simulink model "Residential_grid4"  (R2026a)
settings: Solver=VariableStepAuto  StopTime=365*24*3600
undefined symbols (not defined in the file): evCharge, load1, load2, load3, load4, Solar, Wind
libraries: fl_lib x132, nesl_utility x61
(part 1 of 3)
settings Model: Creator=xiaos  LastModifiedBy=hiro
settings DebuggingCC: SaveWithParameterizedLinksMsg=none
settings SimscapeCC: SimscapeNominalValues="[{\"value\":\"1\",\"unit\":\"A\"},{\"value\":\"1\",\"unit\":\"bar\"},{\"value\":\"1\",\"unit\":\"cm^2\"},{\"value\":\"1\",\"unit\":\"cm^3/s\"},{\"value\":\"1\",\"unit\":\"kJ/kg\"},{\"value\":\"1\",\"unit\":\"kW\"},{\"value\":\"1\",\"unit\":\"l\"},{\"value\":\"1\",\"unit\":\"N\"},{\"value\":\"1\",\"unit\":\"N*m\"},{\"value\":\"1\",\"unit\":\"V\"}]"  SimscapeLogType=none  SimscapeLogDataHistory=5000.0

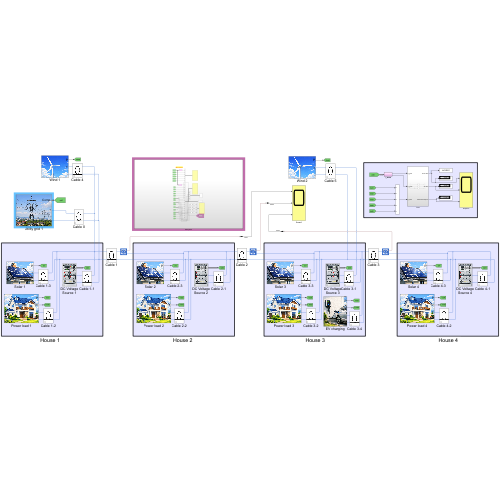
[thumbnail: Simulink's stored preview of the top-level diagram]
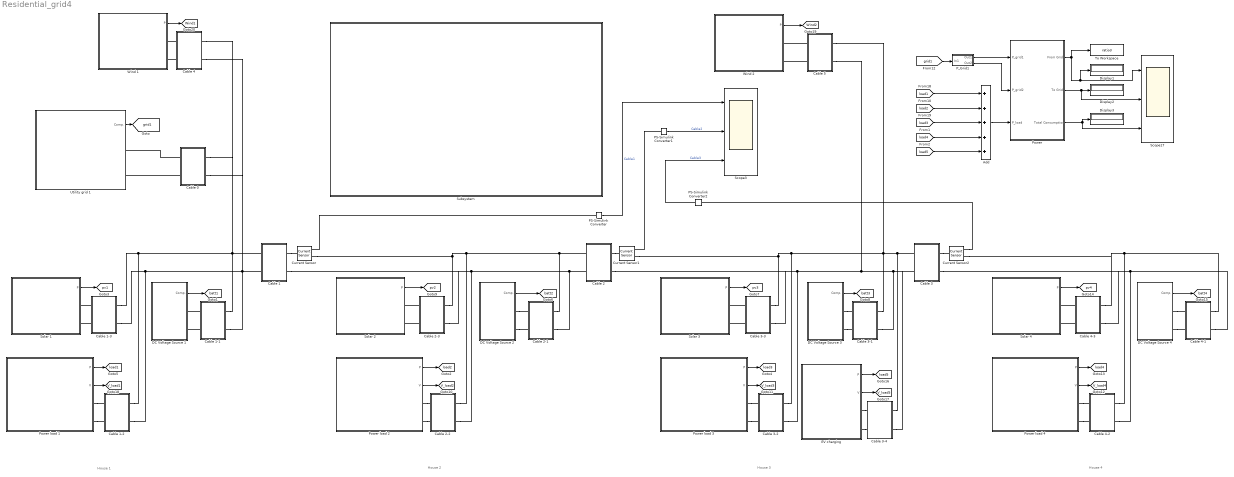
== system Residential_grid4 ==
  note: House 1
  note: House 2
  note: House 3
  note: House 4
  Add : Sum  Inputs=+++++
  Cable 0 : Subsystem  mask{intR=3.01, L=20, SQ=SQ,  rc,  Ampacity}
      mask prompts: intR "Conductor resistance: rc (Ω/km)"; L "Length: L (m)"; SQ "For reference: CV cable constants"
      mask TypeOptions SQ: SQ,  rc,  Ampacity | 2 (mm2),  12 (Ω/km),  28 (A) | 3.5 (mm2),  6.76 (Ω/km),  39 (A) | 5.5 (mm2),  4.34 (Ω/km),  52 (A) | 8 (mm2),  3.01 (Ω/km),   65 (A) | 14 (mm2),  1.71 (Ω/km),  91 (A) | 22 (mm2),  1.08 (Ω/km),  120 (A) | 38 (mm2),  0.626 (Ω/km),  170 (A) | 60 (mm2),  0.397 (Ω/km),  225 (A) | 100 (mm2),  0.239 (Ω/km),  310 (A) | 150 (mm2),  0.16 (Ω/km),  400 (A) | 200 (mm2),  0.121 (Ω/km),  485 (A) | 250 (mm2),  0.0985 (Ω/km),  560 (A) | 325 (mm2),  0.077 (Ω/km),  660 (A)
      mask DialogControl DescTextVar Prompt: 2-Core CV Cable
      mask Display: image('cable_1.png');
  Cable 1 : Subsystem  mask{intR=3.01, L=50, SQ=SQ,  rc,  Ampacity}
      mask prompts: intR "Conductor resistance: rc (Ω/km)"; L "Length: L (m)"; SQ "For reference: CV cable constants"
      mask TypeOptions SQ: SQ,  rc,  Ampacity | 2 (mm2),  12 (Ω/km),  28 (A) | 3.5 (mm2),  6.76 (Ω/km),  39 (A) | 5.5 (mm2),  4.34 (Ω/km),  52 (A) | 8 (mm2),  3.01 (Ω/km),   65 (A) | 14 (mm2),  1.71 (Ω/km),  91 (A) | 22 (mm2),  1.08 (Ω/km),  120 (A) | 38 (mm2),  0.626 (Ω/km),  170 (A) | 60 (mm2),  0.397 (Ω/km),  225 (A) | 100 (mm2),  0.239 (Ω/km),  310 (A) | 150 (mm2),  0.16 (Ω/km),  400 (A) | 200 (mm2),  0.121 (Ω/km),  485 (A) | 250 (mm2),  0.0985 (Ω/km),  560 (A) | 325 (mm2),  0.077 (Ω/km),  660 (A)
      mask DialogControl DescTextVar Prompt: 2-Core CV Cable
      mask Display: image('cable_2.png');
  Cable 1-1 : Subsystem  mask{intR=3.01, L=5, SQ=SQ,  rc,  Ampacity}
      mask prompts: intR "Conductor resistance: rc (Ω/km)"; L "Length: L (m)"; SQ "For reference: CV cable constants"
      mask TypeOptions SQ: SQ,  rc,  Ampacity | 2 (mm2),  12 (Ω/km),  28 (A) | 3.5 (mm2),  6.76 (Ω/km),  39 (A) | 5.5 (mm2),  4.34 (Ω/km),  52 (A) | 8 (mm2),  3.01 (Ω/km),   65 (A) | 14 (mm2),  1.71 (Ω/km),  91 (A) | 22 (mm2),  1.08 (Ω/km),  120 (A) | 38 (mm2),  0.626 (Ω/km),  170 (A) | 60 (mm2),  0.397 (Ω/km),  225 (A) | 100 (mm2),  0.239 (Ω/km),  310 (A) | 150 (mm2),  0.16 (Ω/km),  400 (A) | 200 (mm2),  0.121 (Ω/km),  485 (A) | 250 (mm2),  0.0985 (Ω/km),  560 (A) | 325 (mm2),  0.077 (Ω/km),  660 (A)
      mask DialogControl DescTextVar Prompt: 2-Core CV Cable
      mask Display: image('cable_7.png');
  Cable 1-2 : Subsystem  mask{intR=3.01, L=10, SQ=SQ,  rc,  Ampacity}
      mask prompts: intR "Conductor resistance: rc (Ω/km)"; L "Length: L (m)"; SQ "For reference: CV cable constants"
      mask TypeOptions SQ: SQ,  rc,  Ampacity | 2 (mm2),  12 (Ω/km),  28 (A) | 3.5 (mm2),  6.76 (Ω/km),  39 (A) | 5.5 (mm2),  4.34 (Ω/km),  52 (A) | 8 (mm2),  3.01 (Ω/km),   65 (A) | 14 (mm2),  1.71 (Ω/km),  91 (A) | 22 (mm2),  1.08 (Ω/km),  120 (A) | 38 (mm2),  0.626 (Ω/km),  170 (A) | 60 (mm2),  0.397 (Ω/km),  225 (A) | 100 (mm2),  0.239 (Ω/km),  310 (A) | 150 (mm2),  0.16 (Ω/km),  400 (A) | 200 (mm2),  0.121 (Ω/km),  485 (A) | 250 (mm2),  0.0985 (Ω/km),  560 (A) | 325 (mm2),  0.077 (Ω/km),  660 (A)
      mask DialogControl DescTextVar Prompt: 2-Core CV Cable
      mask Display: image('cable_8.png');
  Cable 1-3 : Subsystem  mask{intR=3.01, L=10, SQ=SQ,  rc,  Ampacity}
      mask prompts: intR "Conductor resistance: rc (Ω/km)"; L "Length: L (m)"; SQ "For reference: CV cable constants"
      mask TypeOptions SQ: SQ,  rc,  Ampacity | 2 (mm2),  12 (Ω/km),  28 (A) | 3.5 (mm2),  6.76 (Ω/km),  39 (A) | 5.5 (mm2),  4.34 (Ω/km),  52 (A) | 8 (mm2),  3.01 (Ω/km),   65 (A) | 14 (mm2),  1.71 (Ω/km),  91 (A) | 22 (mm2),  1.08 (Ω/km),  120 (A) | 38 (mm2),  0.626 (Ω/km),  170 (A) | 60 (mm2),  0.397 (Ω/km),  225 (A) | 100 (mm2),  0.239 (Ω/km),  310 (A) | 150 (mm2),  0.16 (Ω/km),  400 (A) | 200 (mm2),  0.121 (Ω/km),  485 (A) | 250 (mm2),  0.0985 (Ω/km),  560 (A) | 325 (mm2),  0.077 (Ω/km),  660 (A)
      mask DialogControl DescTextVar Prompt: 2-Core CV Cable
      mask Display: image('cable_9.png');
  Cable 2 : Subsystem  mask{intR=3.01, L=50, SQ=SQ,  rc,  Ampacity}
      mask prompts: intR "Conductor resistance: rc (Ω/km)"; L "Length: L (m)"; SQ "For reference: CV cable constants"
      mask TypeOptions SQ: SQ,  rc,  Ampacity | 2 (mm2),  12 (Ω/km),  28 (A) | 3.5 (mm2),  6.76 (Ω/km),  39 (A) | 5.5 (mm2),  4.34 (Ω/km),  52 (A) | 8 (mm2),  3.01 (Ω/km),   65 (A) | 14 (mm2),  1.71 (Ω/km),  91 (A) | 22 (mm2),  1.08 (Ω/km),  120 (A) | 38 (mm2),  0.626 (Ω/km),  170 (A) | 60 (mm2),  0.397 (Ω/km),  225 (A) | 100 (mm2),  0.239 (Ω/km),  310 (A) | 150 (mm2),  0.16 (Ω/km),  400 (A) | 200 (mm2),  0.121 (Ω/km),  485 (A) | 250 (mm2),  0.0985 (Ω/km),  560 (A) | 325 (mm2),  0.077 (Ω/km),  660 (A)
      mask DialogControl DescTextVar Prompt: 2-Core CV Cable
      mask Display: image('cable_3.png');
  Cable 2-1 : Subsystem  mask{intR=3.01, L=5, SQ=SQ,  rc,  Ampacity}
      mask prompts: intR "Conductor resistance: rc (Ω/km)"; L "Length: L (m)"; SQ "For reference: CV cable constants"
      mask TypeOptions SQ: SQ,  rc,  Ampacity | 2 (mm2),  12 (Ω/km),  28 (A) | 3.5 (mm2),  6.76 (Ω/km),  39 (A) | 5.5 (mm2),  4.34 (Ω/km),  52 (A) | 8 (mm2),  3.01 (Ω/km),   65 (A) | 14 (mm2),  1.71 (Ω/km),  91 (A) | 22 (mm2),  1.08 (Ω/km),  120 (A) | 38 (mm2),  0.626 (Ω/km),  170 (A) | 60 (mm2),  0.397 (Ω/km),  225 (A) | 100 (mm2),  0.239 (Ω/km),  310 (A) | 150 (mm2),  0.16 (Ω/km),  400 (A) | 200 (mm2),  0.121 (Ω/km),  485 (A) | 250 (mm2),  0.0985 (Ω/km),  560 (A) | 325 (mm2),  0.077 (Ω/km),  660 (A)
      mask DialogControl DescTextVar Prompt: 2-Core CV Cable
      mask Display: image('cable_10.png');
  Cable 2-2 : Subsystem  mask{intR=3.01, L=10, SQ=SQ,  rc,  Ampacity}
      mask prompts: intR "Conductor resistance: rc (Ω/km)"; L "Length: L (m)"; SQ "For reference: CV cable constants"
      mask TypeOptions SQ: SQ,  rc,  Ampacity | 2 (mm2),  12 (Ω/km),  28 (A) | 3.5 (mm2),  6.76 (Ω/km),  39 (A) | 5.5 (mm2),  4.34 (Ω/km),  52 (A) | 8 (mm2),  3.01 (Ω/km),   65 (A) | 14 (mm2),  1.71 (Ω/km),  91 (A) | 22 (mm2),  1.08 (Ω/km),  120 (A) | 38 (mm2),  0.626 (Ω/km),  170 (A) | 60 (mm2),  0.397 (Ω/km),  225 (A) | 100 (mm2),  0.239 (Ω/km),  310 (A) | 150 (mm2),  0.16 (Ω/km),  400 (A) | 200 (mm2),  0.121 (Ω/km),  485 (A) | 250 (mm2),  0.0985 (Ω/km),  560 (A) | 325 (mm2),  0.077 (Ω/km),  660 (A)
      mask DialogControl DescTextVar Prompt: 2-Core CV Cable
      mask Display: image('cable_11.png');
  Cable 2-3 : Subsystem  mask{intR=3.01, L=10, SQ=SQ,  rc,  Ampacity}
      mask prompts: intR "Conductor resistance: rc (Ω/km)"; L "Length: L (m)"; SQ "For reference: CV cable constants"
      mask TypeOptions SQ: SQ,  rc,  Ampacity | 2 (mm2),  12 (Ω/km),  28 (A) | 3.5 (mm2),  6.76 (Ω/km),  39 (A) | 5.5 (mm2),  4.34 (Ω/km),  52 (A) | 8 (mm2),  3.01 (Ω/km),   65 (A) | 14 (mm2),  1.71 (Ω/km),  91 (A) | 22 (mm2),  1.08 (Ω/km),  120 (A) | 38 (mm2),  0.626 (Ω/km),  170 (A) | 60 (mm2),  0.397 (Ω/km),  225 (A) | 100 (mm2),  0.239 (Ω/km),  310 (A) | 150 (mm2),  0.16 (Ω/km),  400 (A) | 200 (mm2),  0.121 (Ω/km),  485 (A) | 250 (mm2),  0.0985 (Ω/km),  560 (A) | 325 (mm2),  0.077 (Ω/km),  660 (A)
      mask DialogControl DescTextVar Prompt: 2-Core CV Cable
      mask Display: image('cable_12.png');
  Cable 3 : Subsystem  mask{intR=3.01, L=50, SQ=SQ,  rc,  Ampacity}
      mask prompts: intR "Conductor resistance: rc (Ω/km)"; L "Length: L (m)"; SQ "For reference: CV cable constants"
      mask TypeOptions SQ: SQ,  rc,  Ampacity | 2 (mm2),  12 (Ω/km),  28 (A) | 3.5 (mm2),  6.76 (Ω/km),  39 (A) | 5.5 (mm2),  4.34 (Ω/km),  52 (A) | 8 (mm2),  3.01 (Ω/km),   65 (A) | 14 (mm2),  1.71 (Ω/km),  91 (A) | 22 (mm2),  1.08 (Ω/km),  120 (A) | 38 (mm2),  0.626 (Ω/km),  170 (A) | 60 (mm2),  0.397 (Ω/km),  225 (A) | 100 (mm2),  0.239 (Ω/km),  310 (A) | 150 (mm2),  0.16 (Ω/km),  400 (A) | 200 (mm2),  0.121 (Ω/km),  485 (A) | 250 (mm2),  0.0985 (Ω/km),  560 (A) | 325 (mm2),  0.077 (Ω/km),  660 (A)
      mask DialogControl DescTextVar Prompt: 2-Core CV Cable
      mask Display: image('cable_4.png');
  Cable 3-1 : Subsystem  mask{intR=3.01, L=5, SQ=SQ,  rc,  Ampacity}
      mask prompts: intR "Conductor resistance: rc (Ω/km)"; L "Length: L (m)"; SQ "For reference: CV cable constants"
      mask TypeOptions SQ: SQ,  rc,  Ampacity | 2 (mm2),  12 (Ω/km),  28 (A) | 3.5 (mm2),  6.76 (Ω/km),  39 (A) | 5.5 (mm2),  4.34 (Ω/km),  52 (A) | 8 (mm2),  3.01 (Ω/km),   65 (A) | 14 (mm2),  1.71 (Ω/km),  91 (A) | 22 (mm2),  1.08 (Ω/km),  120 (A) | 38 (mm2),  0.626 (Ω/km),  170 (A) | 60 (mm2),  0.397 (Ω/km),  225 (A) | 100 (mm2),  0.239 (Ω/km),  310 (A) | 150 (mm2),  0.16 (Ω/km),  400 (A) | 200 (mm2),  0.121 (Ω/km),  485 (A) | 250 (mm2),  0.0985 (Ω/km),  560 (A) | 325 (mm2),  0.077 (Ω/km),  660 (A)
      mask DialogControl DescTextVar Prompt: 2-Core CV Cable
      mask Display: image('cable_13.png');
  Cable 3-2 : Subsystem  mask{intR=3.01, L=10, SQ=SQ,  rc,  Ampacity}
      mask prompts: intR "Conductor resistance: rc (Ω/km)"; L "Length: L (m)"; SQ "For reference: CV cable constants"
      mask TypeOptions SQ: SQ,  rc,  Ampacity | 2 (mm2),  12 (Ω/km),  28 (A) | 3.5 (mm2),  6.76 (Ω/km),  39 (A) | 5.5 (mm2),  4.34 (Ω/km),  52 (A) | 8 (mm2),  3.01 (Ω/km),   65 (A) | 14 (mm2),  1.71 (Ω/km),  91 (A) | 22 (mm2),  1.08 (Ω/km),  120 (A) | 38 (mm2),  0.626 (Ω/km),  170 (A) | 60 (mm2),  0.397 (Ω/km),  225 (A) | 100 (mm2),  0.239 (Ω/km),  310 (A) | 150 (mm2),  0.16 (Ω/km),  400 (A) | 200 (mm2),  0.121 (Ω/km),  485 (A) | 250 (mm2),  0.0985 (Ω/km),  560 (A) | 325 (mm2),  0.077 (Ω/km),  660 (A)
      mask DialogControl DescTextVar Prompt: 2-Core CV Cable
      mask Display: image('cable_14.png');
  Cable 3-3 : Subsystem  mask{intR=3.01, L=10, SQ=SQ,  rc,  Ampacity}
      mask prompts: intR "Conductor resistance: rc (Ω/km)"; L "Length: L (m)"; SQ "For reference: CV cable constants"
      mask TypeOptions SQ: SQ,  rc,  Ampacity | 2 (mm2),  12 (Ω/km),  28 (A) | 3.5 (mm2),  6.76 (Ω/km),  39 (A) | 5.5 (mm2),  4.34 (Ω/km),  52 (A) | 8 (mm2),  3.01 (Ω/km),   65 (A) | 14 (mm2),  1.71 (Ω/km),  91 (A) | 22 (mm2),  1.08 (Ω/km),  120 (A) | 38 (mm2),  0.626 (Ω/km),  170 (A) | 60 (mm2),  0.397 (Ω/km),  225 (A) | 100 (mm2),  0.239 (Ω/km),  310 (A) | 150 (mm2),  0.16 (Ω/km),  400 (A) | 200 (mm2),  0.121 (Ω/km),  485 (A) | 250 (mm2),  0.0985 (Ω/km),  560 (A) | 325 (mm2),  0.077 (Ω/km),  660 (A)
      mask DialogControl DescTextVar Prompt: 2-Core CV Cable
      mask Display: image('cable_15.png');
  Cable 3-4 : Subsystem  mask{intR=3.01, L=5, SQ=SQ,  rc,  Ampacity}
      mask prompts: intR "Conductor resistance: rc (Ω/km)"; L "Length: L (m)"; SQ "For reference: CV cable constants"
      mask TypeOptions SQ: SQ,  rc,  Ampacity | 2 (mm2),  12 (Ω/km),  28 (A) | 3.5 (mm2),  6.76 (Ω/km),  39 (A) | 5.5 (mm2),  4.34 (Ω/km),  52 (A) | 8 (mm2),  3.01 (Ω/km),   65 (A) | 14 (mm2),  1.71 (Ω/km),  91 (A) | 22 (mm2),  1.08 (Ω/km),  120 (A) | 38 (mm2),  0.626 (Ω/km),  170 (A) | 60 (mm2),  0.397 (Ω/km),  225 (A) | 100 (mm2),  0.239 (Ω/km),  310 (A) | 150 (mm2),  0.16 (Ω/km),  400 (A) | 200 (mm2),  0.121 (Ω/km),  485 (A) | 250 (mm2),  0.0985 (Ω/km),  560 (A) | 325 (mm2),  0.077 (Ω/km),  660 (A)
      mask DialogControl DescTextVar Prompt: 2-Core CV Cable
      mask Display: image('cable_16.png');
  Cable 4 : Subsystem  mask{intR=3.01, L=20, SQ=SQ,  rc,  Ampacity}
      mask prompts: intR "Conductor resistance: rc (Ω/km)"; L "Length: L (m)"; SQ "For reference: CV cable constants"
      mask TypeOptions SQ: SQ,  rc,  Ampacity | 2 (mm2),  12 (Ω/km),  28 (A) | 3.5 (mm2),  6.76 (Ω/km),  39 (A) | 5.5 (mm2),  4.34 (Ω/km),  52 (A) | 8 (mm2),  3.01 (Ω/km),   65 (A) | 14 (mm2),  1.71 (Ω/km),  91 (A) | 22 (mm2),  1.08 (Ω/km),  120 (A) | 38 (mm2),  0.626 (Ω/km),  170 (A) | 60 (mm2),  0.397 (Ω/km),  225 (A) | 100 (mm2),  0.239 (Ω/km),  310 (A) | 150 (mm2),  0.16 (Ω/km),  400 (A) | 200 (mm2),  0.121 (Ω/km),  485 (A) | 250 (mm2),  0.0985 (Ω/km),  560 (A) | 325 (mm2),  0.077 (Ω/km),  660 (A)
      mask DialogControl DescTextVar Prompt: 2-Core CV Cable
      mask Display: image('cable_5.png');
  Cable 4-1 : Subsystem  mask{intR=3.01, L=5, SQ=SQ,  rc,  Ampacity}
      mask prompts: intR "Conductor resistance: rc (Ω/km)"; L "Length: L (m)"; SQ "For reference: CV cable constants"
      mask TypeOptions SQ: SQ,  rc,  Ampacity | 2 (mm2),  12 (Ω/km),  28 (A) | 3.5 (mm2),  6.76 (Ω/km),  39 (A) | 5.5 (mm2),  4.34 (Ω/km),  52 (A) | 8 (mm2),  3.01 (Ω/km),   65 (A) | 14 (mm2),  1.71 (Ω/km),  91 (A) | 22 (mm2),  1.08 (Ω/km),  120 (A) | 38 (mm2),  0.626 (Ω/km),  170 (A) | 60 (mm2),  0.397 (Ω/km),  225 (A) | 100 (mm2),  0.239 (Ω/km),  310 (A) | 150 (mm2),  0.16 (Ω/km),  400 (A) | 200 (mm2),  0.121 (Ω/km),  485 (A) | 250 (mm2),  0.0985 (Ω/km),  560 (A) | 325 (mm2),  0.077 (Ω/km),  660 (A)
      mask DialogControl DescTextVar Prompt: 2-Core CV Cable
      mask Display: image('cable_17.png');
  Cable 4-2 : Subsystem  mask{intR=3.01, L=10, SQ=SQ,  rc,  Ampacity}
      mask prompts: intR "Conductor resistance: rc (Ω/km)"; L "Length: L (m)"; SQ "For reference: CV cable constants"
      mask TypeOptions SQ: SQ,  rc,  Ampacity | 2 (mm2),  12 (Ω/km),  28 (A) | 3.5 (mm2),  6.76 (Ω/km),  39 (A) | 5.5 (mm2),  4.34 (Ω/km),  52 (A) | 8 (mm2),  3.01 (Ω/km),   65 (A) | 14 (mm2),  1.71 (Ω/km),  91 (A) | 22 (mm2),  1.08 (Ω/km),  120 (A) | 38 (mm2),  0.626 (Ω/km),  170 (A) | 60 (mm2),  0.397 (Ω/km),  225 (A) | 100 (mm2),  0.239 (Ω/km),  310 (A) | 150 (mm2),  0.16 (Ω/km),  400 (A) | 200 (mm2),  0.121 (Ω/km),  485 (A) | 250 (mm2),  0.0985 (Ω/km),  560 (A) | 325 (mm2),  0.077 (Ω/km),  660 (A)
      mask DialogControl DescTextVar Prompt: 2-Core CV Cable
      mask Display: image('cable_19.png');
  Cable 4-3 : Subsystem  mask{intR=3.01, L=10, SQ=SQ,  rc,  Ampacity}
      mask prompts: intR "Conductor resistance: rc (Ω/km)"; L "Length: L (m)"; SQ "For reference: CV cable constants"
      mask TypeOptions SQ: SQ,  rc,  Ampacity | 2 (mm2),  12 (Ω/km),  28 (A) | 3.5 (mm2),  6.76 (Ω/km),  39 (A) | 5.5 (mm2),  4.34 (Ω/km),  52 (A) | 8 (mm2),  3.01 (Ω/km),   65 (A) | 14 (mm2),  1.71 (Ω/km),  91 (A) | 22 (mm2),  1.08 (Ω/km),  120 (A) | 38 (mm2),  0.626 (Ω/km),  170 (A) | 60 (mm2),  0.397 (Ω/km),  225 (A) | 100 (mm2),  0.239 (Ω/km),  310 (A) | 150 (mm2),  0.16 (Ω/km),  400 (A) | 200 (mm2),  0.121 (Ω/km),  485 (A) | 250 (mm2),  0.0985 (Ω/km),  560 (A) | 325 (mm2),  0.077 (Ω/km),  660 (A)
      mask DialogControl DescTextVar Prompt: 2-Core CV Cable
      mask Display: image('cable_20.png');
  Cable 5 : Subsystem  mask{intR=3.01, L=20, SQ=SQ,  rc,  Ampacity}
      mask prompts: intR "Conductor resistance: rc (Ω/km)"; L "Length: L (m)"; SQ "For reference: CV cable constants"
      mask TypeOptions SQ: SQ,  rc,  Ampacity | 2 (mm2),  12 (Ω/km),  28 (A) | 3.5 (mm2),  6.76 (Ω/km),  39 (A) | 5.5 (mm2),  4.34 (Ω/km),  52 (A) | 8 (mm2),  3.01 (Ω/km),   65 (A) | 14 (mm2),  1.71 (Ω/km),  91 (A) | 22 (mm2),  1.08 (Ω/km),  120 (A) | 38 (mm2),  0.626 (Ω/km),  170 (A) | 60 (mm2),  0.397 (Ω/km),  225 (A) | 100 (mm2),  0.239 (Ω/km),  310 (A) | 150 (mm2),  0.16 (Ω/km),  400 (A) | 200 (mm2),  0.121 (Ω/km),  485 (A) | 250 (mm2),  0.0985 (Ω/km),  560 (A) | 325 (mm2),  0.077 (Ω/km),  660 (A)
      mask DialogControl DescTextVar Prompt: 2-Core CV Cable
      mask Display: image('cable_6.png');
  Current Sensor : fl_lib/Electrical/Electrical Sensors/Current Sensor
  Current Sensor1 : fl_lib/Electrical/Electrical Sensors/Current Sensor
  Current Sensor2 : fl_lib/Electrical/Electrical Sensors/Current Sensor
  DC Voltage Source 1 : Subsystem  mask{V=380, C_batt=25, SOC_Initial=50, Crg_stop_SoC=95, Crg_rec_SoC=90, Dis_rec_SoC=10, Dis_stop_SoC=5, R=.5}
      mask prompts: V "Terminal voltage (V)"; C_batt "Battery capacity (kWh)"; SOC_Initial "Battery Initial SoC (%)"; Crg_stop_SoC "Charging stop SoC (%)"; Crg_rec_SoC "Charging recovery SoC (%)"; Dis_rec_SoC "Discharge recovery SoC (%)"; Dis_stop_SoC "Discharge stop SoC (%)"; R "Droop parameter (V/A)"
      mask DialogControl DescTextVar Prompt: Battery-powered Voltage Source
      mask Display: image('DC電源装置.png');
  DC Voltage Source 2 : Subsystem  mask{V=380, C_batt=25, SOC_Initial=50, Crg_stop_SoC=95, Crg_rec_SoC=90, Dis_rec_SoC=10, Dis_stop_SoC=5, R=.5}
      mask prompts: V "Terminal voltage (V)"; C_batt "Battery capacity (kWh)"; SOC_Initial "Battery Initial SoC (%)"; Crg_stop_SoC "Charging stop SoC (%)"; Crg_rec_SoC "Charging recovery SoC (%)"; Dis_rec_SoC "Discharge recovery SoC (%)"; Dis_stop_SoC "Discharge stop SoC (%)"; R "Droop parameter (V/A)"
      mask DialogControl DescTextVar Prompt: Battery-powered Voltage Source
      mask Display: image('DC電源装置.png');
  DC Voltage Source 3 : Subsystem  mask{V=380, C_batt=25, SOC_Initial=50, Crg_stop_SoC=95, Crg_rec_SoC=90, Dis_rec_SoC=10, Dis_stop_SoC=5, R=.5}
      mask prompts: V "Terminal voltage (V)"; C_batt "Battery capacity (kWh)"; SOC_Initial "Battery Initial SoC (%)"; Crg_stop_SoC "Charging stop SoC (%)"; Crg_rec_SoC "Charging recovery SoC (%)"; Dis_rec_SoC "Discharge recovery SoC (%)"; Dis_stop_SoC "Discharge stop SoC (%)"; R "Droop parameter (V/A)"
      mask DialogControl DescTextVar Prompt: Battery-powered Voltage Source
      mask Display: image('DC電源装置.png');
  DC Voltage Source 4 : Subsystem  mask{V=380, C_batt=25, SOC_Initial=50, Crg_stop_SoC=95, Crg_rec_SoC=90, Dis_rec_SoC=10, Dis_stop_SoC=5, R=.5}
      mask prompts: V "Terminal voltage (V)"; C_batt "Battery capacity (kWh)"; SOC_Initial "Battery Initial SoC (%)"; Crg_stop_SoC "Charging stop SoC (%)"; Crg_rec_SoC "Charging recovery SoC (%)"; Dis_rec_SoC "Discharge recovery SoC (%)"; Dis_stop_SoC "Discharge stop SoC (%)"; R "Droop parameter (V/A)"
      mask DialogControl DescTextVar Prompt: Battery-powered Voltage Source
      mask Display: image('DC電源装置.png');
  Display1 : Display
  Display2 : Display
  Display3 : Display
  EV charging : Subsystem  mask{data=evCharge, timestep=[0:1:24*3600*365-1]}
      mask prompts: data "Power consumption data"
      mask DialogControl DescGroupVar Prompt: EV Charging
      mask Display: image('EV_Charge_1_1.png');
  PS-Simulink Converter : nesl_utility/PS-Simulink Converter  PhysicalDomain=network_engine_domain  SubClassName=ps_output  LeftPortType=input  RightPortType=output  PseudoPeriodic=off  Frequencies=[]  VectorFormat=inherit  Unit=inherit  AffineConversion=off
  PS-Simulink Converter1 : nesl_utility/PS-Simulink Converter  PhysicalDomain=network_engine_domain  SubClassName=ps_output  LeftPortType=input  RightPortType=output  PseudoPeriodic=off  Frequencies=[]  VectorFormat=inherit  Unit=inherit  AffineConversion=off
  PS-Simulink Converter2 : nesl_utility/PS-Simulink Converter  PhysicalDomain=network_engine_domain  SubClassName=ps_output  LeftPortType=input  RightPortType=output  PseudoPeriodic=off  Frequencies=[]  VectorFormat=inherit  Unit=inherit  AffineConversion=off
  P_Grid1 : Subsystem
  Power : Subsystem
  Power load 1 : Subsystem  mask{data=load1, timestep=[0:1:24*3600*365-1]}
      mask prompts: data "Power consumption data"
      mask DialogControl DescGroupVar Prompt: Power Load
      mask Display: image('House_1_1.png');
  Power load 2 : Subsystem  mask{data=load2, timestep=[0:1:24*3600*365-1]}
      mask prompts: data "Power consumption data"
      mask DialogControl DescGroupVar Prompt: Power Load
      mask Display: image('House_2_1.png');
  Power load 3 : Subsystem  mask{data=load3, timestep=[0:1:24*3600*365-1]}
      mask prompts: data "Power consumption data"
      mask DialogControl DescGroupVar Prompt: Power Load
      mask Display: image('House_3_1.png');
  Power load 4 : Subsystem  mask{data=load4, timestep=[0:1:24*3600*365-1]}
      mask prompts: data "Power consumption data"
      mask DialogControl DescGroupVar Prompt: Power Load
      mask Display: image('House_4_1.png');
  Scope17 : Scope  NumInputPorts=3
      settings: ActiveDisplayYMinimum=-5.5021672722991943E+7  ActiveDisplayYMaximum=8.0414431952663391E+10  YLabel=Accumulated Power (W Sec)  DataLoggingDecimation=60  DataLoggingVariableName=ScopeData17
  Scope3 : Scope  NumInputPorts=3
      settings: ActiveDisplayYMinimum=-29.674233791314766  ActiveDisplayYMaximum=25.267781891936018  YLabel=Current (A)  DataLoggingDecimation=60
  Solar 1 : Subsystem  mask{POA=Solar.POA(:,1), Coef=Solar.Coef(:,1), kw=3.5, eff=100, V_Limit=400, Gain=100, timestep=[0:1:24*3600*365-1]}
      mask prompts: POA "Panel of array irradiance: POA"; Coef "Temperature correction coefficient"; kw "Rated output power (kW)"; eff "Location-based efficiency (%)"; V_Limit "Output curtailment start voltage (V)"; Gain "Overvoltage suppression gain (typ. 500)"
      mask DialogControl DescTextVar Prompt: Solar Power System
      mask Display: image('PV_1.png');
  Solar 2 : Subsystem  mask{POA=Solar.POA(:,2), Coef=Solar.Coef(:,2), kw=3.5, eff=100, V_Limit=400, Gain=100, timestep=[0:1:24*3600*365-1]}
      mask prompts: POA "Panel of array irradiance: POA"; Coef "Temperature correction coefficient"; kw "Rated output power (kW)"; eff "Location-based efficiency (%)"; V_Limit "Output curtailment start voltage (V)"; Gain "Overvoltage suppression gain (typ. 500)"
      mask DialogControl DescTextVar Prompt: Solar Power System
      mask Display: image('PV_1.png');
  Solar 3 : Subsystem  mask{POA=Solar.POA(:,5), Coef=Solar.Coef(:,5), kw=3.5, eff=100, V_Limit=400, Gain=100, timestep=[0:1:24*3600*365-1]}
      mask prompts: POA "Panel of array irradiance: POA"; Coef "Temperature correction coefficient"; kw "Rated output power (kW)"; eff "Location-based efficiency (%)"; V_Limit "Output curtailment start voltage (V)"; Gain "Overvoltage suppression gain (typ. 500)"
      mask DialogControl DescTextVar Prompt: Solar Power System
      mask Display: image('PV_1.png');
  Solar 4 : Subsystem  mask{POA=Solar.POA(:,8), Coef=Solar.Coef(:,8), kw=3.5, eff=100, V_Limit=400, Gain=100, timestep=[0:1:24*3600*365-1]}
      mask prompts: POA "Panel of array irradiance: POA"; Coef "Temperature correction coefficient"; kw "Rated output power (kW)"; eff "Location-based efficiency (%)"; V_Limit "Output curtailment start voltage (V)"; Gain "Overvoltage suppression gain (typ. 500)"
      mask DialogControl DescTextVar Prompt: Solar Power System
      mask Display: image('PV_1.png');
  Subsystem : Subsystem
  To Workspace : ToWorkspace  VariableName=ratio3  SaveFormat=Timeseries  SampleTime=-1
  Utility grid 1 : Subsystem  mask{GotoTag=SoC1, send_start_SoC=85, send_stop_SoC=75, receiv_stop_SoC=25, receiv_start_SoC=15, current=30}
      mask prompts: GotoTag "SoC to be referenced"; send_start_SoC "Power sending start SoC (%)"; send_stop_SoC "Power sending stop SoC (%)"; receiv_stop_SoC "Power receiving stop SoC (%)"; receiv_start_SoC "Power receiving start SoC (%)"; current "Grid import/export current (A)"
      mask TypeOptions GotoTag: From3/GotoTag
      mask DialogControl DescTextVar Prompt: Power exchange with the utility grid
      mask Display: image('Grid.png');
  Wind 1 : Subsystem  mask{P_rate=1000, v_rate=10, v_cutin=2, v_cutout=25, V_Limit=400, Gain=100, timestep=[0:1:24*3600*365-1]}
      mask prompts: P_rate "Rated power generation (W)"; v_rate "Rated wind speed (m/s)"; v_cutin "Cut-in wind speed (m/s)"; v_cutout "Cut-out wind speed (m/s)"; V_Limit "Output curtailment start voltage (V)"; Gain "Overvoltage suppression gain (typ. 500)"
      mask DialogControl DescTextVar Prompt: Wind Power System
      mask Display: image('Windmill_1.png');
  Wind 2 : Subsystem  mask{P_rate=1000, v_rate=10, v_cutin=2, v_cutout=25, V_Limit=400, Gain=100, timestep=[0:1:24*3600*365-1]}
      mask prompts: P_rate "Rated power generation (W)"; v_rate "Rated wind speed (m/s)"; v_cutin "Cut-in wind speed (m/s)"; v_cutout "Cut-out wind speed (m/s)"; V_Limit "Output curtailment start voltage (V)"; Gain "Overvoltage suppression gain (typ. 500)"
      mask DialogControl DescTextVar Prompt: Wind Power System
      mask Display: image('Windmill_1.png');
  tag scope: V_load1=global, V_load2=global, V_load3=global, V_load4=global, V_load5=global, Wind1=global, Wind2=global, batt1=global, batt2=global, batt3=global, batt4=global, grid1=global, load1=global, load2=global, load3=global, load4=global, load5=global, pv1=global, pv2=global, pv3=global, pv4=global
  wires:
  Power load 1/1(P) -> [load1]
  Solar 1/1(P) -> [pv1]
  DC Voltage Source 1/1(Comp.) -> [batt1]
  Power load 1/2(V) -> [V_load1]
  Solar 2/1(P) -> [pv2]
  DC Voltage Source 2/1(Comp.) -> [batt2]
  Power load 2/2(V) -> [V_load2]
  Power load 3/1(P) -> [load3]
  Power load 3/2(V) -> [V_load3]
  DC Voltage Source 3/1(Comp.) -> [batt3]
  Power load 4/1(P) -> [load4]
  Power load 4/2(V) -> [V_load4]
  DC Voltage Source 4/1(Comp.) -> [batt4]
  Power/3(Total Consumption) -> Scope17/3, Display3/1
  [load4] -> Add/4
  [load2] -> Add/2
  Add/1 -> Power/3(P_load)
  [load5] -> Add/5
  Power/2(To Grid) -> Scope17/2, Display2/1
  [load1] -> Add/1
  [load3] -> Add/3
  [grid1] -> P_Grid1/1(In1)
  Power/1(From Grid) -> Display1/1, Scope17/1, To Workspace/1
  Power load 2/1(P) -> [load2]
  EV charging/1(P) -> [load5]
  EV charging/2(V) -> [V_load5]
  PS-Simulink Converter1/1 -> Scope3/2  "Cable2"
  Solar 4/1(P) -> [pv4]
  Utility grid 1/1(Comp.) -> [grid1]
  Wind 1/1(P) -> [Wind1]
  Wind 2/1(P) -> [Wind2]
  Solar 3/1(P) -> [pv3]
  PS-Simulink Converter/1 -> Scope3/1  "Cable1"
  PS-Simulink Converter2/1 -> Scope3/3  "Cable3"
  P_Grid1/1(Out1) -> Power/1(P_grid1)
  P_Grid1/2(Out2) -> Power/2(P_grid2)
  connections:
  Cable 1-3/LConn1 -- Solar 1/RConn1
  Cable 1-3/LConn2 -- Solar 1/RConn2
  Cable 1-1/LConn1 -- DC Voltage Source 1/RConn1
  Cable 1-1/LConn2 -- DC Voltage Source 1/RConn2
  Power load 1/RConn2 -- Cable 1-2/LConn2
  Power load 2/RConn1 -- Cable 2-2/LConn1
  DC Voltage Source 2/RConn1 -- Cable 2-1/LConn1
  Cable 2-3/LConn1 -- Solar 2/RConn1
  DC Voltage Source 2/RConn2 -- Cable 2-1/LConn2
  Cable 2-3/LConn2 -- Solar 2/RConn2
  Power load 2/RConn2 -- Cable 2-2/LConn2
  Cable 3-3/LConn2 -- Solar 3/RConn2
  DC Voltage Source 3/RConn2 -- Cable 3-1/LConn2
  Cable 3-3/LConn1 -- Solar 3/RConn1
  DC Voltage Source 3/RConn1 -- Cable 3-1/LConn1
  Power load 3/RConn2 -- Cable 3-2/LConn2
  Power load 3/RConn1 -- Cable 3-2/LConn1
  Cable 4-1/RConn1 -- Cable 4-2/RConn1 -- Cable 4-3/RConn1 -- Current Sensor2/RConn2
  Cable 4-3/LConn2 -- Solar 4/RConn2
  DC Voltage Source 4/RConn2 -- Cable 4-1/LConn2
  Cable 4-3/LConn1 -- Solar 4/RConn1
  DC Voltage Source 4/RConn1 -- Cable 4-1/LConn1
  Power load 4/RConn2 -- Cable 4-2/LConn2
  Power load 4/RConn1 -- Cable 4-2/LConn1
  Power load 1/RConn1 -- Cable 1-2/LConn1
  Cable 1-1/RConn1 -- Cable 1/LConn1 -- Cable 4/RConn1 -- Cable 0/RConn1 -- Cable 1-3/RConn1 -- Cable 1-2/RConn1
  Cable 1-1/RConn2 -- Cable 1/LConn2 -- Cable 4/RConn2 -- Cable 0/RConn2 -- Cable 1-3/RConn2 -- Cable 1-2/RConn2
  Current Sensor/RConn2 -- Cable 2-3/RConn1 -- Cable 2-2/RConn1 -- Cable 2-1/RConn1 -- Cable 2/LConn1
  Current Sensor1/RConn2 -- Cable 3-3/RConn1 -- Cable 3-2/RConn1 -- Cable 3-1/RConn1 -- Cable 5/RConn1 -- Cable 3-4/RConn1 -- Cable 3/LConn1
  Cable 2-3/RConn2 -- Cable 1/RConn2 -- Cable 2-2/RConn2 -- Cable 2-1/RConn2 -- Cable 2/LConn2
  Cable 3-3/RConn2 -- Cable 2/RConn2 -- Cable 3-2/RConn2 -- Cable 5/RConn2 -- Cable 3-1/RConn2 -- Cable 3-4/RConn2 -- Cable 3/LConn2
  Cable 4-3/RConn2 -- Cable 3/RConn2 -- Cable 4-1/RConn2 -- Cable 4-2/RConn2
  EV charging/RConn1 -- Cable 3-4/LConn1
  EV charging/RConn2 -- Cable 3-4/LConn2
  Cable 1/RConn1 -- Current Sensor/LConn1
  PS-Simulink Converter/LConn1 -- Current Sensor/RConn1
  Cable 2/RConn1 -- Current Sensor1/LConn1
  PS-Simulink Converter1/LConn1 -- Current Sensor1/RConn1
  Cable 3/RConn1 -- Current Sensor2/LConn1
  Current Sensor2/RConn1 -- PS-Simulink Converter2/LConn1
  Cable 0/LConn1 -- Utility grid 1/RConn1
  Cable 0/LConn2 -- Utility grid 1/RConn2
  Cable 5/LConn1 -- Wind 2/RConn1
  Cable 5/LConn2 -- Wind 2/RConn2
  Cable 4/LConn1 -- Wind 1/RConn1
  Cable 4/LConn2 -- Wind 1/RConn2

== system Residential_grid4/Cable 0 ==
  Resistor : fl_lib/Electrical/Electrical Elements/Resistor  R=intR/1000*L Ohm  i_specify=off  i_priority=None  i=0 A  i_nominal_specify=off  i_nominal_value=1  i_nominal_unit=A  v_specify=off  v_priority=None  v=0 V  v_nominal_specify=off  v_nominal_value=1  v_nominal_unit=V
  Resistor1 : fl_lib/Electrical/Electrical Elements/Resistor  R=intR/1000*L Ohm  i_specify=off  i_priority=None  i=0 A  i_nominal_specify=off  i_nominal_value=1  i_nominal_unit=A  v_specify=off  v_priority=None  v=0 V  v_nominal_specify=off  v_nominal_value=1  v_nominal_unit=V
  Series RLC Branch1 : PMIOPort  Side=Left
  Series RLC Branch2 : PMIOPort  Port=2  Side=Right
  Series RLC Branch3 : PMIOPort  Port=3  Side=Left
  Series RLC Branch4 : PMIOPort  Port=4  Side=Right
  connections:
  Series RLC Branch3/RConn1 -- Resistor1/LConn1
  Series RLC Branch2/RConn1 -- Resistor/RConn1
  Series RLC Branch1/RConn1 -- Resistor/LConn1
  Series RLC Branch4/RConn1 -- Resistor1/RConn1

== system Residential_grid4/Cable 1 ==
  Resistor : fl_lib/Electrical/Electrical Elements/Resistor  R=intR/1000*L Ohm  i_specify=off  i_priority=None  i=0 A  i_nominal_specify=off  i_nominal_value=1  i_nominal_unit=A  v_specify=off  v_priority=None  v=0 V  v_nominal_specify=off  v_nominal_value=1  v_nominal_unit=V
  Resistor1 : fl_lib/Electrical/Electrical Elements/Resistor  R=intR/1000*L Ohm  i_specify=off  i_priority=None  i=0 A  i_nominal_specify=off  i_nominal_value=1  i_nominal_unit=A  v_specify=off  v_priority=None  v=0 V  v_nominal_specify=off  v_nominal_value=1  v_nominal_unit=V
  Series RLC Branch1 : PMIOPort  Side=Left
  Series RLC Branch2 : PMIOPort  Port=2  Side=Right
  Series RLC Branch3 : PMIOPort  Port=3  Side=Left
  Series RLC Branch4 : PMIOPort  Port=4  Side=Right
  connections:
  Series RLC Branch3/RConn1 -- Resistor1/LConn1
  Series RLC Branch2/RConn1 -- Resistor/RConn1
  Series RLC Branch1/RConn1 -- Resistor/LConn1
  Series RLC Branch4/RConn1 -- Resistor1/RConn1

== system Residential_grid4/Cable 1-1 ==
  Resistor : fl_lib/Electrical/Electrical Elements/Resistor  R=intR/1000*L Ohm  i_specify=off  i_priority=None  i=0 A  i_nominal_specify=off  i_nominal_value=1  i_nominal_unit=A  v_specify=off  v_priority=None  v=0 V  v_nominal_specify=off  v_nominal_value=1  v_nominal_unit=V
  Resistor1 : fl_lib/Electrical/Electrical Elements/Resistor  R=intR/1000*L Ohm  i_specify=off  i_priority=None  i=0 A  i_nominal_specify=off  i_nominal_value=1  i_nominal_unit=A  v_specify=off  v_priority=None  v=0 V  v_nominal_specify=off  v_nominal_value=1  v_nominal_unit=V
  Series RLC Branch1 : PMIOPort  Side=Left
  Series RLC Branch2 : PMIOPort  Port=2  Side=Right
  Series RLC Branch3 : PMIOPort  Port=3  Side=Left
  Series RLC Branch4 : PMIOPort  Port=4  Side=Right
  connections:
  Series RLC Branch3/RConn1 -- Resistor1/LConn1
  Series RLC Branch2/RConn1 -- Resistor/RConn1
  Series RLC Branch1/RConn1 -- Resistor/LConn1
  Series RLC Branch4/RConn1 -- Resistor1/RConn1

== system Residential_grid4/Cable 1-2 ==
  Resistor : fl_lib/Electrical/Electrical Elements/Resistor  R=intR/1000*L Ohm  i_specify=off  i_priority=None  i=0 A  i_nominal_specify=off  i_nominal_value=1  i_nominal_unit=A  v_specify=off  v_priority=None  v=0 V  v_nominal_specify=off  v_nominal_value=1  v_nominal_unit=V
  Resistor1 : fl_lib/Electrical/Electrical Elements/Resistor  R=intR/1000*L Ohm  i_specify=off  i_priority=None  i=0 A  i_nominal_specify=off  i_nominal_value=1  i_nominal_unit=A  v_specify=off  v_priority=None  v=0 V  v_nominal_specify=off  v_nominal_value=1  v_nominal_unit=V
  Series RLC Branch1 : PMIOPort  Side=Left
  Series RLC Branch2 : PMIOPort  Port=2  Side=Right
  Series RLC Branch3 : PMIOPort  Port=3  Side=Left
  Series RLC Branch4 : PMIOPort  Port=4  Side=Right
  connections:
  Series RLC Branch3/RConn1 -- Resistor1/LConn1
  Series RLC Branch2/RConn1 -- Resistor/RConn1
  Series RLC Branch1/RConn1 -- Resistor/LConn1
  Series RLC Branch4/RConn1 -- Resistor1/RConn1

== system Residential_grid4/Cable 1-3 ==
  Resistor : fl_lib/Electrical/Electrical Elements/Resistor  R=intR/1000*L Ohm  i_specify=off  i_priority=None  i=0 A  i_nominal_specify=off  i_nominal_value=1  i_nominal_unit=A  v_specify=off  v_priority=None  v=0 V  v_nominal_specify=off  v_nominal_value=1  v_nominal_unit=V
  Resistor1 : fl_lib/Electrical/Electrical Elements/Resistor  R=intR/1000*L Ohm  i_specify=off  i_priority=None  i=0 A  i_nominal_specify=off  i_nominal_value=1  i_nominal_unit=A  v_specify=off  v_priority=None  v=0 V  v_nominal_specify=off  v_nominal_value=1  v_nominal_unit=V
  Series RLC Branch1 : PMIOPort  Side=Left
  Series RLC Branch2 : PMIOPort  Port=2  Side=Right
  Series RLC Branch3 : PMIOPort  Port=3  Side=Left
  Series RLC Branch4 : PMIOPort  Port=4  Side=Right
  connections:
  Series RLC Branch3/RConn1 -- Resistor1/LConn1
  Series RLC Branch2/RConn1 -- Resistor/RConn1
  Series RLC Branch1/RConn1 -- Resistor/LConn1
  Series RLC Branch4/RConn1 -- Resistor1/RConn1

== system Residential_grid4/Cable 2 ==
  Resistor : fl_lib/Electrical/Electrical Elements/Resistor  R=intR/1000*L Ohm  i_specify=off  i_priority=None  i=0 A  i_nominal_specify=off  i_nominal_value=1  i_nominal_unit=A  v_specify=off  v_priority=None  v=0 V  v_nominal_specify=off  v_nominal_value=1  v_nominal_unit=V
  Resistor1 : fl_lib/Electrical/Electrical Elements/Resistor  R=intR/1000*L Ohm  i_specify=off  i_priority=None  i=0 A  i_nominal_specify=off  i_nominal_value=1  i_nominal_unit=A  v_specify=off  v_priority=None  v=0 V  v_nominal_specify=off  v_nominal_value=1  v_nominal_unit=V
  Series RLC Branch1 : PMIOPort  Side=Left
  Series RLC Branch2 : PMIOPort  Port=2  Side=Right
  Series RLC Branch3 : PMIOPort  Port=3  Side=Left
  Series RLC Branch4 : PMIOPort  Port=4  Side=Right
  connections:
  Series RLC Branch3/RConn1 -- Resistor1/LConn1
  Series RLC Branch2/RConn1 -- Resistor/RConn1
  Series RLC Branch1/RConn1 -- Resistor/LConn1
  Series RLC Branch4/RConn1 -- Resistor1/RConn1

== system Residential_grid4/Cable 2-1 ==
  Resistor : fl_lib/Electrical/Electrical Elements/Resistor  R=intR/1000*L Ohm  i_specify=off  i_priority=None  i=0 A  i_nominal_specify=off  i_nominal_value=1  i_nominal_unit=A  v_specify=off  v_priority=None  v=0 V  v_nominal_specify=off  v_nominal_value=1  v_nominal_unit=V
  Resistor1 : fl_lib/Electrical/Electrical Elements/Resistor  R=intR/1000*L Ohm  i_specify=off  i_priority=None  i=0 A  i_nominal_specify=off  i_nominal_value=1  i_nominal_unit=A  v_specify=off  v_priority=None  v=0 V  v_nominal_specify=off  v_nominal_value=1  v_nominal_unit=V
  Series RLC Branch1 : PMIOPort  Side=Left
  Series RLC Branch2 : PMIOPort  Port=2  Side=Right
  Series RLC Branch3 : PMIOPort  Port=3  Side=Left
  Series RLC Branch4 : PMIOPort  Port=4  Side=Right
  connections:
  Series RLC Branch3/RConn1 -- Resistor1/LConn1
  Series RLC Branch2/RConn1 -- Resistor/RConn1
  Series RLC Branch1/RConn1 -- Resistor/LConn1
  Series RLC Branch4/RConn1 -- Resistor1/RConn1

== system Residential_grid4/Cable 2-2 ==
  Resistor : fl_lib/Electrical/Electrical Elements/Resistor  R=intR/1000*L Ohm  i_specify=off  i_priority=None  i=0 A  i_nominal_specify=off  i_nominal_value=1  i_nominal_unit=A  v_specify=off  v_priority=None  v=0 V  v_nominal_specify=off  v_nominal_value=1  v_nominal_unit=V
  Resistor1 : fl_lib/Electrical/Electrical Elements/Resistor  R=intR/1000*L Ohm  i_specify=off  i_priority=None  i=0 A  i_nominal_specify=off  i_nominal_value=1  i_nominal_unit=A  v_specify=off  v_priority=None  v=0 V  v_nominal_specify=off  v_nominal_value=1  v_nominal_unit=V
  Series RLC Branch1 : PMIOPort  Side=Left
  Series RLC Branch2 : PMIOPort  Port=2  Side=Right
  Series RLC Branch3 : PMIOPort  Port=3  Side=Left
  Series RLC Branch4 : PMIOPort  Port=4  Side=Right
  connections:
  Series RLC Branch3/RConn1 -- Resistor1/LConn1
  Series RLC Branch2/RConn1 -- Resistor/RConn1
  Series RLC Branch1/RConn1 -- Resistor/LConn1
  Series RLC Branch4/RConn1 -- Resistor1/RConn1

== system Residential_grid4/Cable 2-3 ==
  Resistor : fl_lib/Electrical/Electrical Elements/Resistor  R=intR/1000*L Ohm  i_specify=off  i_priority=None  i=0 A  i_nominal_specify=off  i_nominal_value=1  i_nominal_unit=A  v_specify=off  v_priority=None  v=0 V  v_nominal_specify=off  v_nominal_value=1  v_nominal_unit=V
  Resistor1 : fl_lib/Electrical/Electrical Elements/Resistor  R=intR/1000*L Ohm  i_specify=off  i_priority=None  i=0 A  i_nominal_specify=off  i_nominal_value=1  i_nominal_unit=A  v_specify=off  v_priority=None  v=0 V  v_nominal_specify=off  v_nominal_value=1  v_nominal_unit=V
  Series RLC Branch1 : PMIOPort  Side=Left
  Series RLC Branch2 : PMIOPort  Port=2  Side=Right
  Series RLC Branch3 : PMIOPort  Port=3  Side=Left
  Series RLC Branch4 : PMIOPort  Port=4  Side=Right
  connections:
  Series RLC Branch3/RConn1 -- Resistor1/LConn1
  Series RLC Branch2/RConn1 -- Resistor/RConn1
  Series RLC Branch1/RConn1 -- Resistor/LConn1
  Series RLC Branch4/RConn1 -- Resistor1/RConn1

== system Residential_grid4/Cable 3 ==
  Resistor : fl_lib/Electrical/Electrical Elements/Resistor  R=intR/1000*L Ohm  i_specify=off  i_priority=None  i=0 A  i_nominal_specify=off  i_nominal_value=1  i_nominal_unit=A  v_specify=off  v_priority=None  v=0 V  v_nominal_specify=off  v_nominal_value=1  v_nominal_unit=V
  Resistor1 : fl_lib/Electrical/Electrical Elements/Resistor  R=intR/1000*L Ohm  i_specify=off  i_priority=None  i=0 A  i_nominal_specify=off  i_nominal_value=1  i_nominal_unit=A  v_specify=off  v_priority=None  v=0 V  v_nominal_specify=off  v_nominal_value=1  v_nominal_unit=V
  Series RLC Branch1 : PMIOPort  Side=Left
  Series RLC Branch2 : PMIOPort  Port=2  Side=Right
  Series RLC Branch3 : PMIOPort  Port=3  Side=Left
  Series RLC Branch4 : PMIOPort  Port=4  Side=Right
  connections:
  Series RLC Branch3/RConn1 -- Resistor1/LConn1
  Series RLC Branch2/RConn1 -- Resistor/RConn1
  Series RLC Branch1/RConn1 -- Resistor/LConn1
  Series RLC Branch4/RConn1 -- Resistor1/RConn1

== system Residential_grid4/Cable 3-1 ==
  Resistor : fl_lib/Electrical/Electrical Elements/Resistor  R=intR/1000*L Ohm  i_specify=off  i_priority=None  i=0 A  i_nominal_specify=off  i_nominal_value=1  i_nominal_unit=A  v_specify=off  v_priority=None  v=0 V  v_nominal_specify=off  v_nominal_value=1  v_nominal_unit=V
  Resistor1 : fl_lib/Electrical/Electrical Elements/Resistor  R=intR/1000*L Ohm  i_specify=off  i_priority=None  i=0 A  i_nominal_specify=off  i_nominal_value=1  i_nominal_unit=A  v_specify=off  v_priority=None  v=0 V  v_nominal_specify=off  v_nominal_value=1  v_nominal_unit=V
  Series RLC Branch1 : PMIOPort  Side=Left
  Series RLC Branch2 : PMIOPort  Port=2  Side=Right
  Series RLC Branch3 : PMIOPort  Port=3  Side=Left
  Series RLC Branch4 : PMIOPort  Port=4  Side=Right
  connections:
  Series RLC Branch3/RConn1 -- Resistor1/LConn1
  Series RLC Branch2/RConn1 -- Resistor/RConn1
  Series RLC Branch1/RConn1 -- Resistor/LConn1
  Series RLC Branch4/RConn1 -- Resistor1/RConn1

== system Residential_grid4/Cable 3-2 ==
  Resistor : fl_lib/Electrical/Electrical Elements/Resistor  R=intR/1000*L Ohm  i_specify=off  i_priority=None  i=0 A  i_nominal_specify=off  i_nominal_value=1  i_nominal_unit=A  v_specify=off  v_priority=None  v=0 V  v_nominal_specify=off  v_nominal_value=1  v_nominal_unit=V
  Resistor1 : fl_lib/Electrical/Electrical Elements/Resistor  R=intR/1000*L Ohm  i_specify=off  i_priority=None  i=0 A  i_nominal_specify=off  i_nominal_value=1  i_nominal_unit=A  v_specify=off  v_priority=None  v=0 V  v_nominal_specify=off  v_nominal_value=1  v_nominal_unit=V
  Series RLC Branch1 : PMIOPort  Side=Left
  Series RLC Branch2 : PMIOPort  Port=2  Side=Right
  Series RLC Branch3 : PMIOPort  Port=3  Side=Left
  Series RLC Branch4 : PMIOPort  Port=4  Side=Right
  connections:
  Series RLC Branch3/RConn1 -- Resistor1/LConn1
  Series RLC Branch2/RConn1 -- Resistor/RConn1
  Series RLC Branch1/RConn1 -- Resistor/LConn1
  Series RLC Branch4/RConn1 -- Resistor1/RConn1

== system Residential_grid4/Cable 3-3 ==
  Resistor : fl_lib/Electrical/Electrical Elements/Resistor  R=intR/1000*L Ohm  i_specify=off  i_priority=None  i=0 A  i_nominal_specify=off  i_nominal_value=1  i_nominal_unit=A  v_specify=off  v_priority=None  v=0 V  v_nominal_specify=off  v_nominal_value=1  v_nominal_unit=V
  Resistor1 : fl_lib/Electrical/Electrical Elements/Resistor  R=intR/1000*L Ohm  i_specify=off  i_priority=None  i=0 A  i_nominal_specify=off  i_nominal_value=1  i_nominal_unit=A  v_specify=off  v_priority=None  v=0 V  v_nominal_specify=off  v_nominal_value=1  v_nominal_unit=V
  Series RLC Branch1 : PMIOPort  Side=Left
  Series RLC Branch2 : PMIOPort  Port=2  Side=Right
  Series RLC Branch3 : PMIOPort  Port=3  Side=Left
  Series RLC Branch4 : PMIOPort  Port=4  Side=Right
  connections:
  Series RLC Branch3/RConn1 -- Resistor1/LConn1
  Series RLC Branch2/RConn1 -- Resistor/RConn1
  Series RLC Branch1/RConn1 -- Resistor/LConn1
  Series RLC Branch4/RConn1 -- Resistor1/RConn1

== system Residential_grid4/Cable 3-4 ==
  Resistor : fl_lib/Electrical/Electrical Elements/Resistor  R=intR/1000*L Ohm  i_specify=off  i_priority=None  i=0 A  i_nominal_specify=off  i_nominal_value=1  i_nominal_unit=A  v_specify=off  v_priority=None  v=0 V  v_nominal_specify=off  v_nominal_value=1  v_nominal_unit=V
  Resistor1 : fl_lib/Electrical/Electrical Elements/Resistor  R=intR/1000*L Ohm  i_specify=off  i_priority=None  i=0 A  i_nominal_specify=off  i_nominal_value=1  i_nominal_unit=A  v_specify=off  v_priority=None  v=0 V  v_nominal_specify=off  v_nominal_value=1  v_nominal_unit=V
  Series RLC Branch1 : PMIOPort  Side=Left
  Series RLC Branch2 : PMIOPort  Port=2  Side=Right
  Series RLC Branch3 : PMIOPort  Port=3  Side=Left
  Series RLC Branch4 : PMIOPort  Port=4  Side=Right
  connections:
  Series RLC Branch3/RConn1 -- Resistor1/LConn1
  Series RLC Branch2/RConn1 -- Resistor/RConn1
  Series RLC Branch1/RConn1 -- Resistor/LConn1
  Series RLC Branch4/RConn1 -- Resistor1/RConn1

== system Residential_grid4/Cable 4 ==
  Resistor : fl_lib/Electrical/Electrical Elements/Resistor  R=intR/1000*L Ohm  i_specify=off  i_priority=None  i=0 A  i_nominal_specify=off  i_nominal_value=1  i_nominal_unit=A  v_specify=off  v_priority=None  v=0 V  v_nominal_specify=off  v_nominal_value=1  v_nominal_unit=V
  Resistor1 : fl_lib/Electrical/Electrical Elements/Resistor  R=intR/1000*L Ohm  i_specify=off  i_priority=None  i=0 A  i_nominal_specify=off  i_nominal_value=1  i_nominal_unit=A  v_specify=off  v_priority=None  v=0 V  v_nominal_specify=off  v_nominal_value=1  v_nominal_unit=V
  Series RLC Branch1 : PMIOPort  Side=Left
  Series RLC Branch2 : PMIOPort  Port=2  Side=Right
  Series RLC Branch3 : PMIOPort  Port=3  Side=Left
  Series RLC Branch4 : PMIOPort  Port=4  Side=Right
  connections:
  Series RLC Branch3/RConn1 -- Resistor1/LConn1
  Series RLC Branch2/RConn1 -- Resistor/RConn1
  Series RLC Branch1/RConn1 -- Resistor/LConn1
  Series RLC Branch4/RConn1 -- Resistor1/RConn1

== system Residential_grid4/Cable 4-1 ==
  Resistor : fl_lib/Electrical/Electrical Elements/Resistor  R=intR/1000*L Ohm  i_specify=off  i_priority=None  i=0 A  i_nominal_specify=off  i_nominal_value=1  i_nominal_unit=A  v_specify=off  v_priority=None  v=0 V  v_nominal_specify=off  v_nominal_value=1  v_nominal_unit=V
  Resistor1 : fl_lib/Electrical/Electrical Elements/Resistor  R=intR/1000*L Ohm  i_specify=off  i_priority=None  i=0 A  i_nominal_specify=off  i_nominal_value=1  i_nominal_unit=A  v_specify=off  v_priority=None  v=0 V  v_nominal_specify=off  v_nominal_value=1  v_nominal_unit=V
  Series RLC Branch1 : PMIOPort  Side=Left
  Series RLC Branch2 : PMIOPort  Port=2  Side=Right
  Series RLC Branch3 : PMIOPort  Port=3  Side=Left
  Series RLC Branch4 : PMIOPort  Port=4  Side=Right
  connections:
  Series RLC Branch3/RConn1 -- Resistor1/LConn1
  Series RLC Branch2/RConn1 -- Resistor/RConn1
  Series RLC Branch1/RConn1 -- Resistor/LConn1
  Series RLC Branch4/RConn1 -- Resistor1/RConn1

== system Residential_grid4/Cable 4-2 ==
  Resistor : fl_lib/Electrical/Electrical Elements/Resistor  R=intR/1000*L Ohm  i_specify=off  i_priority=None  i=0 A  i_nominal_specify=off  i_nominal_value=1  i_nominal_unit=A  v_specify=off  v_priority=None  v=0 V  v_nominal_specify=off  v_nominal_value=1  v_nominal_unit=V
  Resistor1 : fl_lib/Electrical/Electrical Elements/Resistor  R=intR/1000*L Ohm  i_specify=off  i_priority=None  i=0 A  i_nominal_specify=off  i_nominal_value=1  i_nominal_unit=A  v_specify=off  v_priority=None  v=0 V  v_nominal_specify=off  v_nominal_value=1  v_nominal_unit=V
  Series RLC Branch1 : PMIOPort  Side=Left
  Series RLC Branch2 : PMIOPort  Port=2  Side=Right
  Series RLC Branch3 : PMIOPort  Port=3  Side=Left
  Series RLC Branch4 : PMIOPort  Port=4  Side=Right
  connections:
  Series RLC Branch3/RConn1 -- Resistor1/LConn1
  Series RLC Branch2/RConn1 -- Resistor/RConn1
  Series RLC Branch1/RConn1 -- Resistor/LConn1
  Series RLC Branch4/RConn1 -- Resistor1/RConn1

== system Residential_grid4/Cable 4-3 ==
  Resistor : fl_lib/Electrical/Electrical Elements/Resistor  R=intR/1000*L Ohm  i_specify=off  i_priority=None  i=0 A  i_nominal_specify=off  i_nominal_value=1  i_nominal_unit=A  v_specify=off  v_priority=None  v=0 V  v_nominal_specify=off  v_nominal_value=1  v_nominal_unit=V
  Resistor1 : fl_lib/Electrical/Electrical Elements/Resistor  R=intR/1000*L Ohm  i_specify=off  i_priority=None  i=0 A  i_nominal_specify=off  i_nominal_value=1  i_nominal_unit=A  v_specify=off  v_priority=None  v=0 V  v_nominal_specify=off  v_nominal_value=1  v_nominal_unit=V
  Series RLC Branch1 : PMIOPort  Side=Left
  Series RLC Branch2 : PMIOPort  Port=2  Side=Right
  Series RLC Branch3 : PMIOPort  Port=3  Side=Left
  Series RLC Branch4 : PMIOPort  Port=4  Side=Right
  connections:
  Series RLC Branch3/RConn1 -- Resistor1/LConn1
  Series RLC Branch2/RConn1 -- Resistor/RConn1
  Series RLC Branch1/RConn1 -- Resistor/LConn1
  Series RLC Branch4/RConn1 -- Resistor1/RConn1

== system Residential_grid4/Cable 5 ==
  Resistor : fl_lib/Electrical/Electrical Elements/Resistor  R=intR/1000*L Ohm  i_specify=off  i_priority=None  i=0 A  i_nominal_specify=off  i_nominal_value=1  i_nominal_unit=A  v_specify=off  v_priority=None  v=0 V  v_nominal_specify=off  v_nominal_value=1  v_nominal_unit=V
  Resistor1 : fl_lib/Electrical/Electrical Elements/Resistor  R=intR/1000*L Ohm  i_specify=off  i_priority=None  i=0 A  i_nominal_specify=off  i_nominal_value=1  i_nominal_unit=A  v_specify=off  v_priority=None  v=0 V  v_nominal_specify=off  v_nominal_value=1  v_nominal_unit=V
  Series RLC Branch1 : PMIOPort  Side=Left
  Series RLC Branch2 : PMIOPort  Port=2  Side=Right
  Series RLC Branch3 : PMIOPort  Port=3  Side=Left
  Series RLC Branch4 : PMIOPort  Port=4  Side=Right
  connections:
  Series RLC Branch3/RConn1 -- Resistor1/LConn1
  Series RLC Branch2/RConn1 -- Resistor/RConn1
  Series RLC Branch1/RConn1 -- Resistor/LConn1
  Series RLC Branch4/RConn1 -- Resistor1/RConn1
